simulink model "glider_attitude_backstepping_R2018b"  (R2018b)
settings: Solver=VariableStepAuto  StartTime=0.0  StopTime=Param.Tend  MinStep=0.001  RelTol=1e-3
InitFcn:
  | glider_init;
StopFcn:
  | glider_show_data;
undefined symbols (not defined in the file or in its folder): Param
settings Model: SimulationMode=accelerator  EnablePacing=on  PacingRate=1000  Creator=joaom  LastModifiedBy=Bruno
settings DataIOCC: ReturnWorkspaceOutputs=on

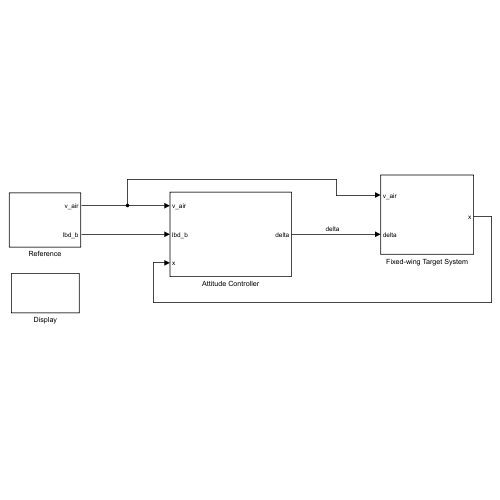
[thumbnail: Simulink's stored preview of the top-level diagram]
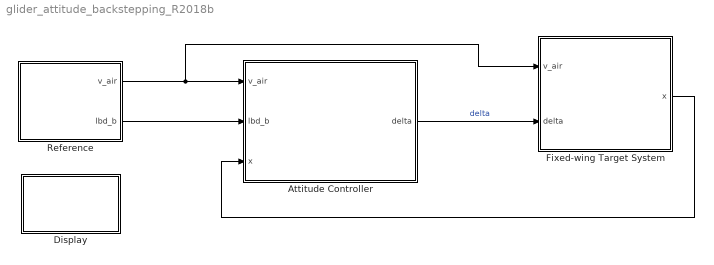
== system glider_attitude_backstepping_R2018b ==
  Attitude Controller : Subsystem
  Display : Subsystem
  Fixed-wing Target System : Subsystem
  Reference : Subsystem
  wires:
  Attitude Controller/1(delta) -> Fixed-wing Target System/2(delta)  "delta"
  Fixed-wing Target System/1(x) -> Attitude Controller/3(x)
  Reference/2(lbd_b) -> Attitude Controller/2(lbd_b)
  Reference/1(v_air) -> Fixed-wing Target System/1(v_air), Attitude Controller/1(v_air)

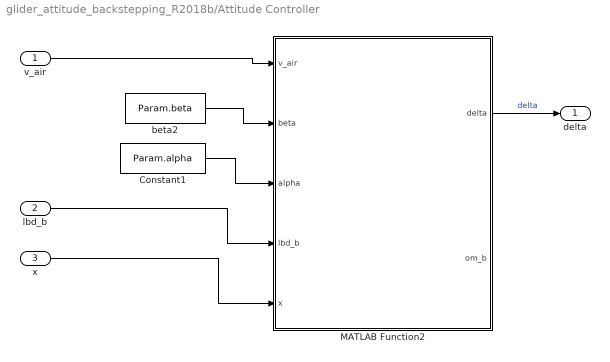
== system glider_attitude_backstepping_R2018b/Attitude Controller ==
  v_air : Inport
  lbd_b : Inport  Port=2
  x : Inport  Port=3
  Constant1 : Constant  Value=Param.alpha
  MATLAB Function2 : MATLAB Function  TreatAsAtomicUnit=on
  beta2 : Constant  Value=Param.beta
  delta : Outport
  wires:
  lbd_b/1 -> MATLAB Function2/4(lbd_b)
  x/1 -> MATLAB Function2/5(x)
  beta2/1 -> MATLAB Function2/2(beta)
  Constant1/1 -> MATLAB Function2/3(alpha)
  v_air/1 -> MATLAB Function2/1(v_air)
  MATLAB Function2/1(delta) -> delta/1  "delta"

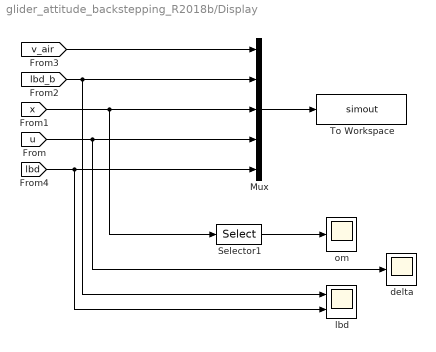
== system glider_attitude_backstepping_R2018b/Display ==
  Mux : Mux  Inputs=5
  Selector1 : Selector  InputPortWidth=12  IndexOptions=Index vector (dialog)  Indices=[10:12]  OutputSizes=1
  To Workspace : ToWorkspace  VariableName=simout  SaveFormat=Structure With Time  SampleTime=-1
  delta : Scope
  lbd : Scope  NumInputPorts=2
  om : Scope
  wires:
  [x] -> Selector1/1, Mux/3
  [u] -> delta/1, Mux/4
  [lbd_b] -> lbd/1, Mux/2
  Mux/1 -> To Workspace/1
  Selector1/1 -> om/1
  [lbd] -> lbd/2, Mux/5
  [v_air] -> Mux/1

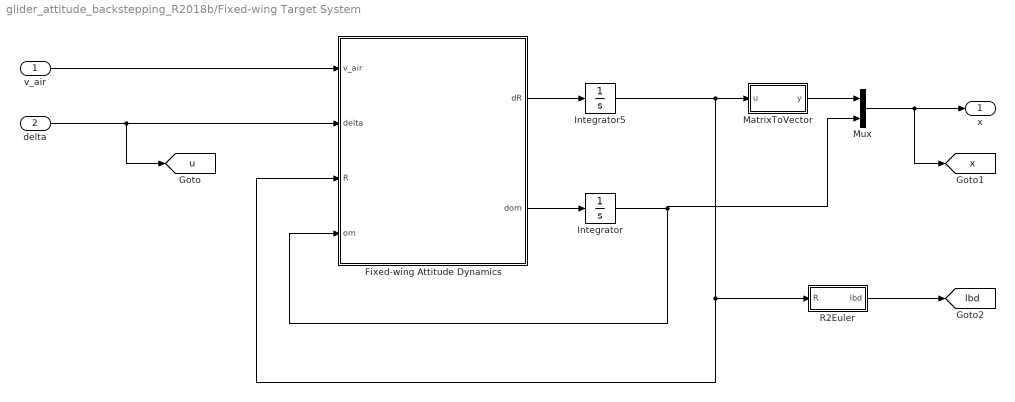
== system glider_attitude_backstepping_R2018b/Fixed-wing Target System ==
  v_air : Inport
  delta : Inport  Port=2
  Fixed-wing Attitude Dynamics : MATLAB Function  TreatAsAtomicUnit=on
  Integrator : Integrator  InitialCondition=Param.om0
  Integrator5 : Integrator  InitialCondition=Param.R0
  MatrixToVector : MATLAB Function  TreatAsAtomicUnit=on
  Mux : Mux  Inputs=2
  R2Euler : MATLAB Function  TreatAsAtomicUnit=on
  x : Outport
  tag scope: lbd=global, u=global, x=global
  wires:
  Fixed-wing Attitude Dynamics/2(dom) -> Integrator/1
  Fixed-wing Attitude Dynamics/1(dR) -> Integrator5/1
  Integrator5/1 -> R2Euler/1(R), Fixed-wing Attitude Dynamics/3(R), MatrixToVector/1(u)
  delta/1 -> [u], Fixed-wing Attitude Dynamics/2(delta)
  Mux/1 -> [x], x/1
  Integrator/1 -> Mux/2, Fixed-wing Attitude Dynamics/4(om)
  v_air/1 -> Fixed-wing Attitude Dynamics/1(v_air)
  R2Euler/1(lbd) -> [lbd]
  MatrixToVector/1(y) -> Mux/1

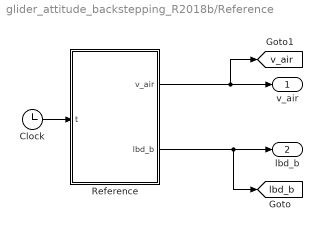
== system glider_attitude_backstepping_R2018b/Reference ==
  Clock : Clock
  Reference : MATLAB Function  TreatAsAtomicUnit=on
  v_air : Outport
  lbd_b : Outport  Port=2
  tag scope: lbd_b=global, v_air=global
  wires:
  Reference/2(lbd_b) -> [lbd_b], lbd_b/1
  Reference/1(v_air) -> [v_air], v_air/1
  Clock/1 -> Reference/1(t)

== matlab function glider_attitude_backstepping_R2018b/Fixed-wing Target System/Fixed-wing Attitude Dynamics ==
  data: v_air input; delta input size=3; R input; om input size=3; dR output; Param parameter; dom output
function [dR,dom] = dynamics_att(v_air, delta, R, om, Param)

    [dR,dom] = fw_drone_att_dyn(v_air,R,om,delta,Param);

end

== matlab function glider_attitude_backstepping_R2018b/Reference/Reference ==
  data: t input; v_air output; lbd_b output; Param parameter
function [v_air,lbd_b] = get_ref(t,Param)
    
    [v_air,lbd_b] = gen_reference(t,Param);

end

== matlab function glider_attitude_backstepping_R2018b/Fixed-wing Target System/MatrixToVector ==
  data: u input; y output
function y = fcn(u)

y = u(:);

== matlab function glider_attitude_backstepping_R2018b/Fixed-wing Target System/R2Euler ==
  data: R input; lbd output
function lbd = fcn(R)

lbd = R2Euler(R);

== matlab function glider_attitude_backstepping_R2018b/Attitude Controller/MATLAB Function2 ==
  data: v_air input; beta input; alpha input; lbd_b input; x input; delta output; Param parameter; om_b output size=3
function [delta, om_b] = deltas(v_air, beta, alpha, lbd_b, x, Param)

    [delta, om_b] = att_controller(v_air, beta, alpha, lbd_b, x, Param);

end
